simulink model "EMG_Gripper_System_enhanced"  (R2025a)
settings: Solver=FixedStepDiscrete  StartTime=0  StopTime=10  FixedStep=0.005  RelTol=1e-3
settings Model: Creator=mahdi  LastModifiedBy=mahdi

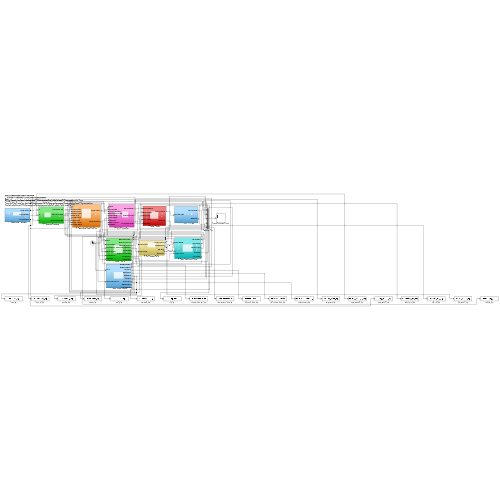
[thumbnail: Simulink's stored preview of the top-level diagram]
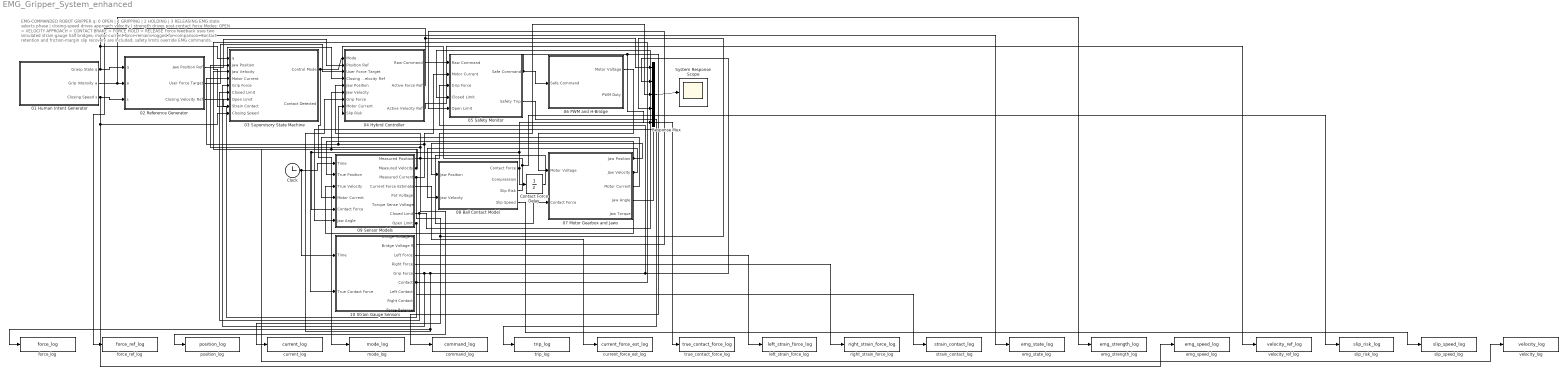
== system EMG_Gripper_System_enhanced ==
  note: EMG-COMMANDED ROBOT GRIPPER
      | q: 0 OPEN | 1 GRIPPING | 2 HOLDING | 3 RELEASING
      | EMG state selects phase | closing-speed drives approach velocity | strength drives post-contact force
      | Modes: OPEN > VELOCITY APPROACH > CONTACT BRAKE > FORCE HOLD > RELEASE
      | Force feedback uses two simulated strain-gauge half bridges; motor-current force remains logged for comparison.
      | Contact retention and friction-margin slip recovery are included; safety limits override EMG commands.
  01 Human Intent Generator : Subsystem
  02 Reference Generator : Subsystem
  03 Supervisory State Machine : Subsystem
  04 Hybrid Controller : Subsystem
  05 Safety Monitor : Subsystem
  06 PWM and H-Bridge : Subsystem
  07 Motor Gearbox and Jaws : Subsystem
  08 Ball Contact Model : Subsystem
  09 Sensor Models : Subsystem
  10 Strain Gauge Sensors : Subsystem
  Clock : Clock
  Contact Force Delay : UnitDelay  SampleTime=0.005  HasFrameUpgradeWarning=on
  Response Mux : Mux  Inputs=5
  System Response Scope : Scope
      settings: ActiveDisplayYMinimum=-2.4655819338309253  ActiveDisplayYMaximum=16.516915530641974
  command_log : ToWorkspace  VariableName=command_log  SaveFormat=Timeseries  SampleTime=-1
  current_force_est_log : ToWorkspace  VariableName=current_force_est_log  SaveFormat=Timeseries  SampleTime=-1
  current_log : ToWorkspace  VariableName=current_log  SaveFormat=Timeseries  SampleTime=-1
  emg_speed_log : ToWorkspace  VariableName=emg_speed_log  SaveFormat=Timeseries  SampleTime=-1
  emg_state_log : ToWorkspace  VariableName=emg_state_log  SaveFormat=Timeseries  SampleTime=-1
  emg_strength_log : ToWorkspace  VariableName=emg_strength_log  SaveFormat=Timeseries  SampleTime=-1
  force_log : ToWorkspace  VariableName=force_log  SaveFormat=Timeseries  SampleTime=-1
  force_ref_log : ToWorkspace  VariableName=force_ref_log  SaveFormat=Timeseries  SampleTime=-1
  left_strain_force_log : ToWorkspace  VariableName=left_strain_force_log  SaveFormat=Timeseries  SampleTime=-1
  mode_log : ToWorkspace  VariableName=mode_log  SaveFormat=Timeseries  SampleTime=-1
  position_log : ToWorkspace  VariableName=position_log  SaveFormat=Timeseries  SampleTime=-1
  right_strain_force_log : ToWorkspace  VariableName=right_strain_force_log  SaveFormat=Timeseries  SampleTime=-1
  slip_risk_log : ToWorkspace  VariableName=slip_risk_log  SaveFormat=Timeseries  SampleTime=-1
  slip_speed_log : ToWorkspace  VariableName=slip_speed_log  SaveFormat=Timeseries  SampleTime=-1
  strain_contact_log : ToWorkspace  VariableName=strain_contact_log  SaveFormat=Timeseries  SampleTime=-1
  trip_log : ToWorkspace  VariableName=trip_log  SaveFormat=Timeseries  SampleTime=-1
  true_contact_force_log : ToWorkspace  VariableName=true_contact_force_log  SaveFormat=Timeseries  SampleTime=-1
  velocity_log : ToWorkspace  VariableName=velocity_log  SaveFormat=Timeseries  SampleTime=-1
  velocity_ref_log : ToWorkspace  VariableName=velocity_ref_log  SaveFormat=Timeseries  SampleTime=-1
  wires:
  01 Human Intent Generator/1(Grasp State q) -> 03 Supervisory State Machine/1(q), emg_state_log/1, 02 Reference Generator/1(q)
  01 Human Intent Generator/2(Grip Intensity a) -> 02 Reference Generator/2(a), emg_strength_log/1
  01 Human Intent Generator/3(Closing Speed s) -> 03 Supervisory State Machine/9(Closing Speed), emg_speed_log/1, 02 Reference Generator/3(s)
  02 Reference Generator/1(Jaw Position Ref) -> 04 Hybrid Controller/2(Position Ref)
  02 Reference Generator/2(User Force Target) -> 04 Hybrid Controller/3(User Force Target)
  02 Reference Generator/3(Closing Velocity Ref) -> 04 Hybrid Controller/4(Closing Velocity Ref)
  03 Supervisory State Machine/1(Control Mode) -> 04 Hybrid Controller/1(Mode), mode_log/1
  04 Hybrid Controller/1(Raw Command) -> 05 Safety Monitor/1(Raw Command)
  05 Safety Monitor/1(Safe Command) -> command_log/1, Response Mux/5, 06 PWM and H-Bridge/1(Safe Command)
  06 PWM and H-Bridge/1(Motor Voltage) -> 07 Motor Gearbox and Jaws/1(Motor Voltage)
  07 Motor Gearbox and Jaws/1(Jaw Position) -> 08 Ball Contact Model/1(Jaw Position), 09 Sensor Models/2(True Position)
  07 Motor Gearbox and Jaws/2(Jaw Velocity) -> 08 Ball Contact Model/2(Jaw Velocity), 09 Sensor Models/3(True Velocity)
  08 Ball Contact Model/1(Contact Force) -> 09 Sensor Models/5(Contact Force), 10 Strain Gauge Sensors/2(True Contact Force), true_contact_force_log/1, Contact Force Delay/1
  Contact Force Delay/1 -> 07 Motor Gearbox and Jaws/2(Contact Force)
  Clock/1 -> 09 Sensor Models/1(Time), 10 Strain Gauge Sensors/1(Time)
  07 Motor Gearbox and Jaws/3(Motor Current) -> 09 Sensor Models/4(Motor Current)
  07 Motor Gearbox and Jaws/4(Jaw Angle) -> 09 Sensor Models/6(Jaw Angle)
  09 Sensor Models/1(Measured Position) -> Response Mux/3, 03 Supervisory State Machine/2(Jaw Position), 04 Hybrid Controller/5(Jaw Position), position_log/1
  09 Sensor Models/2(Measured Velocity) -> 04 Hybrid Controller/6(Jaw Velocity), velocity_log/1, 03 Supervisory State Machine/3(Jaw Velocity)
  09 Sensor Models/3(Measured Current) -> current_log/1, Response Mux/4, 03 Supervisory State Machine/4(Motor Current), 04 Hybrid Controller/8(Motor Current), 05 Safety Monitor/2(Motor Current)
  10 Strain Gauge Sensors/5(Grip Force) -> Response Mux/2, 05 Safety Monitor/3(Grip Force), force_log/1, 04 Hybrid Controller/7(Grip Force), 03 Supervisory State Machine/5(Grip Force)
  09 Sensor Models/7(Closed Limit) -> 03 Supervisory State Machine/6(Closed Limit), 05 Safety Monitor/4(Closed Limit)
  09 Sensor Models/8(Open Limit) -> 03 Supervisory State Machine/7(Open Limit), 05 Safety Monitor/5(Open Limit)
  10 Strain Gauge Sensors/6(Contact) -> 03 Supervisory State Machine/8(Strain Contact), strain_contact_log/1
  08 Ball Contact Model/3(Slip Risk) -> 04 Hybrid Controller/9(Slip Risk), slip_risk_log/1
  04 Hybrid Controller/2(Active Force Ref) -> force_ref_log/1, Response Mux/1
  05 Safety Monitor/2(Safety Trip) -> trip_log/1
  09 Sensor Models/4(Current Force Estimate) -> current_force_est_log/1
  10 Strain Gauge Sensors/3(Left Force) -> left_strain_force_log/1
  10 Strain Gauge Sensors/4(Right Force) -> right_strain_force_log/1
  04 Hybrid Controller/3(Active Velocity Ref) -> velocity_ref_log/1
  08 Ball Contact Model/4(Slip Speed) -> slip_speed_log/1
  Response Mux/1 -> System Response Scope/1

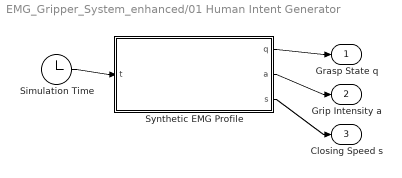
== system EMG_Gripper_System_enhanced/01 Human Intent Generator ==
  Simulation Time : Clock
  Synthetic EMG Profile : MATLAB Function  TreatAsAtomicUnit=on
  Grasp State q : Outport
  Grip Intensity a : Outport  Port=2
  Closing Speed s : Outport  Port=3
  wires:
  Simulation Time/1 -> Synthetic EMG Profile/1(t)
  Synthetic EMG Profile/1(q) -> Grasp State q/1
  Synthetic EMG Profile/2(a) -> Grip Intensity a/1
  Synthetic EMG Profile/3(s) -> Closing Speed s/1

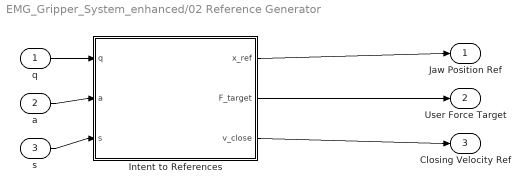
== system EMG_Gripper_System_enhanced/02 Reference Generator ==
  q : Inport
  a : Inport  Port=2
  s : Inport  Port=3
  Intent to References : MATLAB Function  TreatAsAtomicUnit=on
  Jaw Position Ref : Outport
  User Force Target : Outport  Port=2
  Closing Velocity Ref : Outport  Port=3
  wires:
  q/1 -> Intent to References/1(q)
  a/1 -> Intent to References/2(a)
  s/1 -> Intent to References/3(s)
  Intent to References/1(x_ref) -> Jaw Position Ref/1
  Intent to References/2(F_target) -> User Force Target/1
  Intent to References/3(v_close) -> Closing Velocity Ref/1

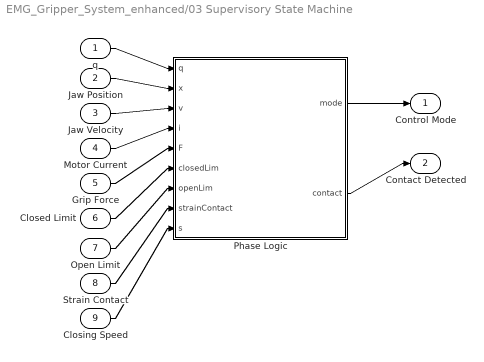
== system EMG_Gripper_System_enhanced/03 Supervisory State Machine ==
  q : Inport
  Jaw Position : Inport  Port=2
  Jaw Velocity : Inport  Port=3
  Motor Current : Inport  Port=4
  Grip Force : Inport  Port=5
  Closed Limit : Inport  Port=6
  Open Limit : Inport  Port=7
  Strain Contact : Inport  Port=8
  Closing Speed : Inport  Port=9
  Phase Logic : MATLAB Function  TreatAsAtomicUnit=on
  Control Mode : Outport
  Contact Detected : Outport  Port=2
  wires:
  q/1 -> Phase Logic/1(q)
  Jaw Position/1 -> Phase Logic/2(x)
  Jaw Velocity/1 -> Phase Logic/3(v)
  Motor Current/1 -> Phase Logic/4(i)
  Grip Force/1 -> Phase Logic/5(F)
  Closed Limit/1 -> Phase Logic/6(closedLim)
  Open Limit/1 -> Phase Logic/7(openLim)
  Strain Contact/1 -> Phase Logic/8(strainContact)
  Closing Speed/1 -> Phase Logic/9(s)
  Phase Logic/1(mode) -> Control Mode/1
  Phase Logic/2(contact) -> Contact Detected/1

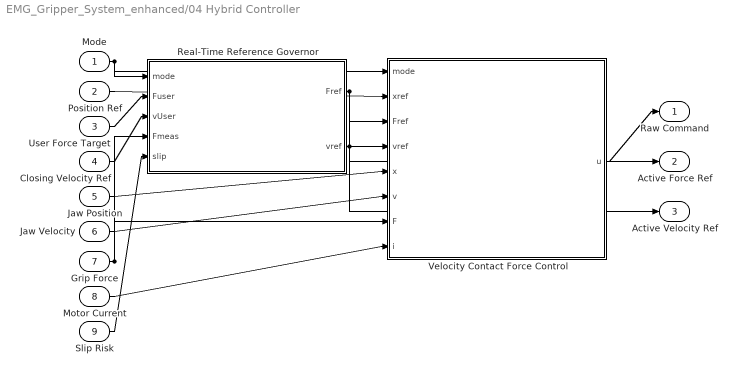
== system EMG_Gripper_System_enhanced/04 Hybrid Controller ==
  Mode : Inport
  Position Ref : Inport  Port=2
  User Force Target : Inport  Port=3
  Closing Velocity Ref : Inport  Port=4
  Jaw Position : Inport  Port=5
  Jaw Velocity : Inport  Port=6
  Grip Force : Inport  Port=7
  Motor Current : Inport  Port=8
  Slip Risk : Inport  Port=9
  Real-Time Reference Governor : MATLAB Function  TreatAsAtomicUnit=on
  Velocity Contact Force Control : MATLAB Function  TreatAsAtomicUnit=on
  Raw Command : Outport
  Active Force Ref : Outport  Port=2
  Active Velocity Ref : Outport  Port=3
  wires:
  Mode/1 -> Real-Time Reference Governor/1(mode), Velocity Contact Force Control/1(mode)
  User Force Target/1 -> Real-Time Reference Governor/2(Fuser)
  Closing Velocity Ref/1 -> Real-Time Reference Governor/3(vUser)
  Grip Force/1 -> Real-Time Reference Governor/4(Fmeas), Velocity Contact Force Control/7(F)
  Slip Risk/1 -> Real-Time Reference Governor/5(slip)
  Position Ref/1 -> Velocity Contact Force Control/2(xref)
  Real-Time Reference Governor/1(Fref) -> Velocity Contact Force Control/3(Fref), Active Force Ref/1
  Real-Time Reference Governor/2(vref) -> Velocity Contact Force Control/4(vref), Active Velocity Ref/1
  Jaw Position/1 -> Velocity Contact Force Control/5(x)
  Jaw Velocity/1 -> Velocity Contact Force Control/6(v)
  Motor Current/1 -> Velocity Contact Force Control/8(i)
  Velocity Contact Force Control/1(u) -> Raw Command/1

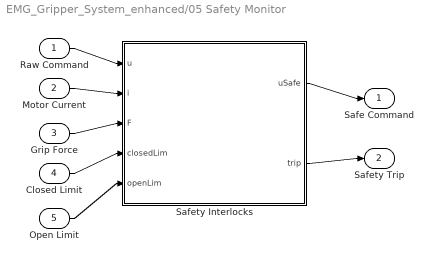
== system EMG_Gripper_System_enhanced/05 Safety Monitor ==
  Raw Command : Inport
  Motor Current : Inport  Port=2
  Grip Force : Inport  Port=3
  Closed Limit : Inport  Port=4
  Open Limit : Inport  Port=5
  Safety Interlocks : MATLAB Function  TreatAsAtomicUnit=on
  Safe Command : Outport
  Safety Trip : Outport  Port=2
  wires:
  Raw Command/1 -> Safety Interlocks/1(u)
  Motor Current/1 -> Safety Interlocks/2(i)
  Grip Force/1 -> Safety Interlocks/3(F)
  Closed Limit/1 -> Safety Interlocks/4(closedLim)
  Open Limit/1 -> Safety Interlocks/5(openLim)
  Safety Interlocks/1(uSafe) -> Safe Command/1
  Safety Interlocks/2(trip) -> Safety Trip/1

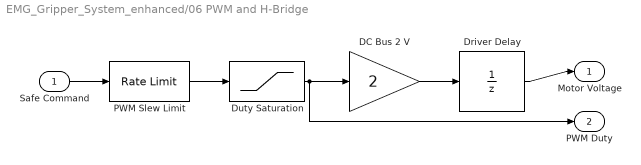
== system EMG_Gripper_System_enhanced/06 PWM and H-Bridge ==
  Safe Command : Inport
  DC Bus 2 V : Gain  Gain=2
  Driver Delay : UnitDelay  SampleTime=0.005  HasFrameUpgradeWarning=on
  Duty Saturation : Saturate  UpperLimit=1  LowerLimit=-1
  PWM Slew Limit : RateLimiter  RisingSlewLimit=6  FallingSlewLimit=-6  SampleTimeMode=inherited
  Motor Voltage : Outport
  PWM Duty : Outport  Port=2
  wires:
  Safe Command/1 -> PWM Slew Limit/1
  PWM Slew Limit/1 -> Duty Saturation/1
  Duty Saturation/1 -> DC Bus 2 V/1, PWM Duty/1
  DC Bus 2 V/1 -> Driver Delay/1
  Driver Delay/1 -> Motor Voltage/1

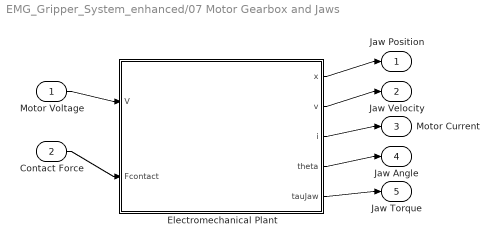
== system EMG_Gripper_System_enhanced/07 Motor Gearbox and Jaws ==
  Motor Voltage : Inport
  Contact Force : Inport  Port=2
  Electromechanical Plant : MATLAB Function  TreatAsAtomicUnit=on
  Jaw Position : Outport
  Jaw Velocity : Outport  Port=2
  Motor Current : Outport  Port=3
  Jaw Angle : Outport  Port=4
  Jaw Torque : Outport  Port=5
  wires:
  Motor Voltage/1 -> Electromechanical Plant/1(V)
  Contact Force/1 -> Electromechanical Plant/2(Fcontact)
  Electromechanical Plant/1(x) -> Jaw Position/1
  Electromechanical Plant/2(v) -> Jaw Velocity/1
  Electromechanical Plant/3(i) -> Motor Current/1
  Electromechanical Plant/4(theta) -> Jaw Angle/1
  Electromechanical Plant/5(tauJaw) -> Jaw Torque/1

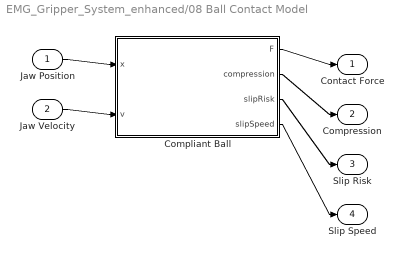
== system EMG_Gripper_System_enhanced/08 Ball Contact Model ==
  Jaw Position : Inport
  Jaw Velocity : Inport  Port=2
  Compliant Ball : MATLAB Function  TreatAsAtomicUnit=on
  Contact Force : Outport
  Compression : Outport  Port=2
  Slip Risk : Outport  Port=3
  Slip Speed : Outport  Port=4
  wires:
  Jaw Position/1 -> Compliant Ball/1(x)
  Jaw Velocity/1 -> Compliant Ball/2(v)
  Compliant Ball/1(F) -> Contact Force/1
  Compliant Ball/2(compression) -> Compression/1
  Compliant Ball/3(slipRisk) -> Slip Risk/1
  Compliant Ball/4(slipSpeed) -> Slip Speed/1

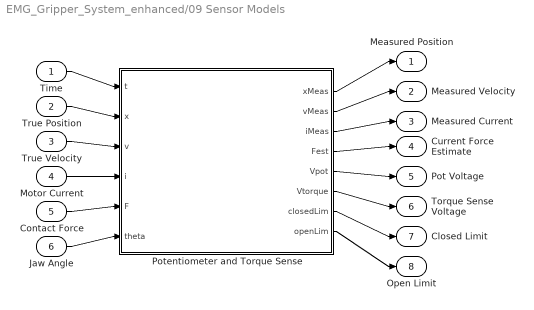
== system EMG_Gripper_System_enhanced/09 Sensor Models ==
  Time : Inport
  True Position : Inport  Port=2
  True Velocity : Inport  Port=3
  Motor Current : Inport  Port=4
  Contact Force : Inport  Port=5
  Jaw Angle : Inport  Port=6
  Potentiometer and Torque Sense : MATLAB Function  TreatAsAtomicUnit=on
  Measured Position : Outport
  Measured Velocity : Outport  Port=2
  Measured Current : Outport  Port=3
  Current Force Estimate : Outport  Port=4
  Pot Voltage : Outport  Port=5
  Torque Sense Voltage : Outport  Port=6
  Closed Limit : Outport  Port=7
  Open Limit : Outport  Port=8
  wires:
  Time/1 -> Potentiometer and Torque Sense/1(t)
  True Position/1 -> Potentiometer and Torque Sense/2(x)
  True Velocity/1 -> Potentiometer and Torque Sense/3(v)
  Motor Current/1 -> Potentiometer and Torque Sense/4(i)
  Contact Force/1 -> Potentiometer and Torque Sense/5(F)
  Jaw Angle/1 -> Potentiometer and Torque Sense/6(theta)
  Potentiometer and Torque Sense/1(xMeas) -> Measured Position/1
  Potentiometer and Torque Sense/2(vMeas) -> Measured Velocity/1
  Potentiometer and Torque Sense/3(iMeas) -> Measured Current/1
  Potentiometer and Torque Sense/4(Fest) -> Current Force Estimate/1
  Potentiometer and Torque Sense/5(Vpot) -> Pot Voltage/1
  Potentiometer and Torque Sense/6(Vtorque) -> Torque Sense Voltage/1
  Potentiometer and Torque Sense/7(closedLim) -> Closed Limit/1
  Potentiometer and Torque Sense/8(openLim) -> Open Limit/1

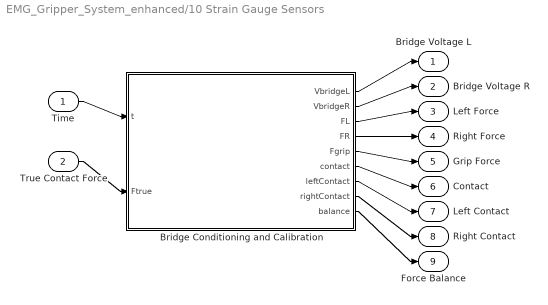
== system EMG_Gripper_System_enhanced/10 Strain Gauge Sensors ==
  Time : Inport
  True Contact Force : Inport  Port=2
  Bridge Conditioning and Calibration : MATLAB Function  TreatAsAtomicUnit=on
  Bridge Voltage L : Outport
  Bridge Voltage R : Outport  Port=2
  Left Force : Outport  Port=3
  Right Force : Outport  Port=4
  Grip Force : Outport  Port=5
  Contact : Outport  Port=6
  Left Contact : Outport  Port=7
  Right Contact : Outport  Port=8
  Force Balance : Outport  Port=9
  wires:
  Time/1 -> Bridge Conditioning and Calibration/1(t)
  True Contact Force/1 -> Bridge Conditioning and Calibration/2(Ftrue)
  Bridge Conditioning and Calibration/1(VbridgeL) -> Bridge Voltage L/1
  Bridge Conditioning and Calibration/2(VbridgeR) -> Bridge Voltage R/1
  Bridge Conditioning and Calibration/3(FL) -> Left Force/1
  Bridge Conditioning and Calibration/4(FR) -> Right Force/1
  Bridge Conditioning and Calibration/5(Fgrip) -> Grip Force/1
  Bridge Conditioning and Calibration/6(contact) -> Contact/1
  Bridge Conditioning and Calibration/7(leftContact) -> Left Contact/1
  Bridge Conditioning and Calibration/8(rightContact) -> Right Contact/1
  Bridge Conditioning and Calibration/9(balance) -> Force Balance/1

== matlab function EMG_Gripper_System_enhanced/08 Ball Contact Model/Compliant Ball ==
  data: x input; F output; v input; compression output; slipRisk output; slipSpeed output
function [F,compression,slipRisk,slipSpeed] = fcn(x,v)
% 32 mm Kelvin-Voigt object plus a simple gravity/friction slip model.
persistent grasped vy
if isempty(grasped), grasped=0; vy=0; end
Ts=0.005; diameter=0.032; k=4500; c=35; mass=0.060; mu=0.25; g=9.81;
compression=max(diameter-x,0);
if compression > 0
    F=max(k*compression+c*max(-v,0),0);
else
    F=0;
end
F=min(F,124.6);
if ~grasped && F>0.5, grasped=1; end
if grasped
    support=2*mu*F; deficit=max(mass*g-support,0);
    if deficit>0, vy=vy+Ts*deficit/mass; else, vy=max(vy-6*Ts,0); end
else
    vy=0;
end
slipRisk=double(grasped && (vy>0.002 || 2*mu*F<1.10*mass*g));
slipSpeed=vy;

== matlab function EMG_Gripper_System_enhanced/09 Sensor Models/Potentiometer and Torque Sense ==
  data: t input; xMeas output; x input; v input; i input; F input; theta input; vMeas output; iMeas output; Fest output; Vpot output; Vtorque output; closedLim output; openLim output
function [xMeas,vMeas,iMeas,Fest,Vpot,Vtorque,closedLim,openLim] = fcn(t,x,v,i,F,theta)
% Datasheet sensor relations with deterministic low-level ripple.
Vexc=5; Rtorque=1; Kt=0.31*0.00706155; Ng=49.3; Nj=50; eta=0.50; r=0.03175;
xMeas=min(max(x + 2e-5*sin(2*pi*17*t),0),0.0508);
vMeas=v; iMeas=i + 5e-4*sin(2*pi*23*t);
Vpot=(Vexc/3)*(theta/(pi/2));
Vtorque=abs(iMeas)*Rtorque;
thetaEff=max(theta,7*pi/180);
Fest=min(abs(eta*Ng*Nj*Kt*iMeas)/(r*sin(thetaEff)),124.6);
if F < 0.5, Fest=0; end
closedLim = double(x <= 2e-4); openLim = double(x >= (0.0508-2e-4));

== matlab function EMG_Gripper_System_enhanced/10 Strain Gauge Sensors/Bridge Conditioning and Calibration ==
  data: t input; VbridgeL output; Ftrue input; VbridgeR output; FL output; FR output; Fgrip output; contact output; leftContact output; rightContact output; balance output
function [VbridgeL,VbridgeR,FL,FR,Fgrip,contact,leftContact,rightContact,balance] = fcn(t,Ftrue)
% Two bending half bridges, amplifier/ADC, calibration, filtering and hysteresis.
persistent fLstate fRstate contactState
if isempty(fLstate), fLstate=0; fRstate=0; contactState=0; end
Ts=0.005; tau=0.005; alpha=Ts/(tau+Ts);
E=69e9; b=0.015; h=0.003; Lg=0.045; GF=2.1; Vex=3.3; Gamp=100;
Vfs=3.3; levels=4095; lsb=Vfs/levels;
Keps=6*Lg/(E*b*h^2);
Ftrue=max(Ftrue,0);
asym=0.01*sin(2*pi*0.6*t);
FtrueL=Ftrue*(1+asym); FtrueR=Ftrue*(1-asym);
epsL=Keps*FtrueL; epsR=Keps*FtrueR;
VbridgeL=Vex*GF*epsL/2; VbridgeR=Vex*GF*epsR/2;
noiseL=0.0015*sin(2*pi*31*t)+0.0003*sin(2*pi*0.08*t);
noiseR=0.0015*sin(2*pi*29*t+0.7)-0.0003*sin(2*pi*0.08*t);
VadcL=min(max(Gamp*VbridgeL+noiseL,0),Vfs);
VadcR=min(max(Gamp*VbridgeR+noiseR,0),Vfs);
VadcL=round(VadcL/lsb)*lsb; VadcR=round(VadcR/lsb)*lsb;
Kv=Gamp*Vex*GF*Keps/2;
FrawL=VadcL/Kv; FrawR=VadcR/Kv;
fLstate=fLstate+alpha*(FrawL-fLstate);
fRstate=fRstate+alpha*(FrawR-fRstate);
FL=max(fLstate,0); FR=max(fRstate,0); Fgrip=(FL+FR)/2;
leftContact=double(FL>0.30); rightContact=double(FR>0.30);
if contactState<0.5 && Fgrip>0.30, contactState=1; end
if contactState>0.5 && Fgrip<0.12, contactState=0; end
contact=contactState; balance=FL-FR;

== matlab function EMG_Gripper_System_enhanced/02 Reference Generator/Intent to References ==
  data: q input; x_ref output; a input; s input; F_target output; v_close output
function [x_ref,F_target,v_close] = fcn(q,a,s)
% Separate references: strength controls force; closing-speed controls approach.
x_max = 0.0508;
a = min(max(a,0),1); s = min(max(s,0),1);
if q == 0 || q == 3
    x_ref = x_max; F_target = 0;
else
    x_ref = 0; F_target = 5 + 13*a^1.35;
end
% 7-22 mm/s approach range. Preview starts motion before the state edge;
% contact braking and force limits remain the authoritative safety layer.
v_close = -(0.007 + 0.015*s);
if s < 0.02 && q == 0, v_close = 0; end

== matlab function EMG_Gripper_System_enhanced/01 Human Intent Generator/Synthetic EMG Profile ==
  data: t input; q output; a output; s output
function [q,a,s] = fcn(t)
% q: state, a: normalized strength, s: previewed normalized closing speed.
if t < 0.45
    q = 0; a = 0; s = 0;
elseif t < 0.75
    q = 0; a = 0; s = 0.65*(t-0.45)/0.30;
elseif t < 1
    q = 0; a = 0; s = 0.65;
elseif t < 2
    q = 1; a = 0.5*(t-1); s = 0.65;
elseif t < 5
    q = 2; a = 0.5; s = 0;
elseif t < 6
    q = 2; a = 0.5 + 0.3*(t-5); s = 0;
elseif t < 8
    q = 2; a = 0.8; s = 0;
elseif t < 9
    q = 3; a = 0.8*(9-t); s = 0;
else
    q = 0; a = 0; s = 0;
end

== matlab function EMG_Gripper_System_enhanced/03 Supervisory State Machine/Phase Logic ==
  data: q input; mode output; x input; v input; i input; F input; closedLim input; openLim input; strainContact input; s input; contact output
function [mode,contact] = fcn(q,x,v,i,F,closedLim,openLim,strainContact,s)
% 0 OPEN, 1 VELOCITY APPROACH, 2 CONTACT BRAKE, 3 FORCE HOLD, 4 RELEASE.
persistent contactLatch brakeTicks previewTicks
if isempty(contactLatch), contactLatch=0; brakeTicks=0; previewTicks=0; end
rawContact=(strainContact>0.5)||(F>0.30)||((abs(i)>0.10)&&(abs(v)<0.002));
if s>0.10, previewTicks=min(previewTicks+1,20); else, previewTicks=max(previewTicks-1,0); end
previewReady=(previewTicks>=3);
if (q==0 && s<0.05) || q==3
    contactLatch=0; brakeTicks=0;
elseif ~contactLatch && (rawContact || closedLim)
    contactLatch=1; brakeTicks=10;
end
if q==3
    mode=4;
elseif q==0 && ~previewReady
    mode=0;
elseif ~contactLatch
    mode=1;
elseif brakeTicks>0
    mode=2; brakeTicks=brakeTicks-1;
else
    mode=3;
end
if openLim && q==0 && ~previewReady, mode=0; end
contact=double(contactLatch);

== matlab function EMG_Gripper_System_enhanced/04 Hybrid Controller/Real-Time Reference Governor ==
  data: mode input; Fref output; Fuser input; vUser input; Fmeas input; slip input; vref output
function [Fref,vref] = fcn(mode,Fuser,vUser,Fmeas,slip)
persistent fState slipBoost prevMode
if isempty(fState), fState=0; slipBoost=0; prevMode=-1; end
Ts=0.005; Fsafe=18;
if mode==3 && slip>0.5, slipBoost=min(slipBoost+6*Ts,3); else, slipBoost=max(slipBoost-0.8*Ts,0); end
Fcmd=min(max(Fuser+slipBoost,0),Fsafe);
if mode==1
    Fref=0; fState=0; vref=vUser;
elseif mode==2
    fState=min(max(Fmeas,0.5),max(Fcmd,0.5)); Fref=fState; vref=0;
elseif mode==3
    if prevMode==2, fState=min(max(Fmeas,0.5),Fcmd); end
    d=Fcmd-fState;
    if d>=0, step=min(d,25*Ts); else, step=max(d,-40*Ts); end
    fState=fState+step; Fref=fState; vref=0;
else
    fState=0; Fref=0; vref=0;
end
prevMode=mode;

== matlab function EMG_Gripper_System_enhanced/04 Hybrid Controller/Velocity Contact Force Control ==
  data: mode input; u output; xref input; Fref input; vref input; x input; v input; F input; i input
function u = fcn(mode,xref,Fref,vref,x,v,F,i)
% Multimode 5 ms controller. Positive command opens jaws.
persistent iF iV prevMode prevF dFf
if isempty(iF), iF=0; iV=0; prevMode=-1; prevF=0; dFf=0; end
Ts=0.005; dF=(F-prevF)/Ts; dFf=0.75*dFf+0.25*dF;
if mode~=3, iF=0; end
if mode~=1, iV=0; end
if mode==0 || mode==4
    u=28*(xref-x)-1.5*v;
elseif mode==1
    eV=vref-v; iVc=min(max(iV+Ts*eV,-0.04),0.04);
    uUnsat=25*vref+12*eV+12*iVc; u=min(max(uUnsat,-0.7),0.15);
    if abs(uUnsat)<0.7, iV=iVc; end
elseif mode==2
    % Short active brake: dissipate approach energy without fully unloading contact.
    u=min(max(-16*v+0.00045*max(dFf,0),0),0.28);
    if F<0.8, u=min(u,0.05); end
else
    e=Fref-F; iFc=min(max(iF+Ts*e,-15),15);
    uUnsat=-(0.012*e+0.060*iFc)-8*v+0.00035*dFf;
    Ffloor=max(1.2,0.35*Fref);
    if F<Ffloor
        u=min(max(uUnsat,-0.7),0);
        if F<0.5*Ffloor, u=min(u,-0.08); end
    else
        u=min(max(uUnsat,-0.7),0.08);
    end
    if uUnsat>-0.7 && uUnsat<0.08, iF=iFc; end
end
u=min(max(u,-1),1); prevMode=mode; prevF=F;

== matlab function EMG_Gripper_System_enhanced/05 Safety Monitor/Safety Interlocks ==
  data: u input; uSafe output; i input; F input; closedLim input; openLim input; trip output
function [uSafe,trip] = fcn(u,i,F,closedLim,openLim)
% 70% of the 2 V stall current and 70% of 178 N datasheet peak.
Imax = 0.70*(2/8.5);
Fmax = 0.70*178;
% A 0.7 duty cap on the 2 V bus guarantees <=70% stall current.
uSafe = min(max(u,-0.7),0.7); trip = 0;
if ((abs(i) > 1.02*Imax) && (sign(uSafe)==sign(i))) || (F >= Fmax && uSafe < 0)
    uSafe = 0; trip = 1;
end
if closedLim && uSafe < -0.02, uSafe = 0; trip = 1; end
if openLim && uSafe > 0.02, uSafe = 0; trip = 1; end
if ~isfinite(uSafe), uSafe = 0; trip = 1; end

== matlab function EMG_Gripper_System_enhanced/07 Motor Gearbox and Jaws/Electromechanical Plant ==
  data: V input; x output; Fcontact input; v output; i output; theta output; tauJaw output
function [x,v,i,theta,tauJaw] = fcn(V,Fcontact)
% Discrete nonlinear gripper plant. Outputs are pre-update states.
persistent th w
if isempty(th), th = pi/2; w = 0; end
Ts=0.005; R=8.5; Kt=0.31*0.00706155; Ke=Kt;
Ng=49.3; Nj=50; eta=0.50; J=0.12; B=0.40;
r=0.03175; xMax=0.0508;
x = xMax*th/(pi/2); v = xMax*w/(pi/2); theta = th;
i = min(max((V-Ke*Ng*w)/R,-0.5),0.5);
tauJaw = eta*Ng*Nj*Kt*i;
thetaEff=max(th,7*pi/180);
tauContact = max(Fcontact,0)*r*sin(thetaEff);
tauNet = tauJaw + tauContact - B*w;
wNew = w + Ts*tauNet/J;
thNew = th + Ts*wNew;
if thNew <= 0, thNew=0; wNew=max(wNew,0); end
if thNew >= pi/2, thNew=pi/2; wNew=min(wNew,0); end
th=thNew; w=wNew;
